simulink model "aurora1_adcs_1axis"  (R2026a)
settings: Solver=VariableStepAuto  StopTime=20.0
settings Model: Creator=chancellordelk  LastModifiedBy=chancellordelk

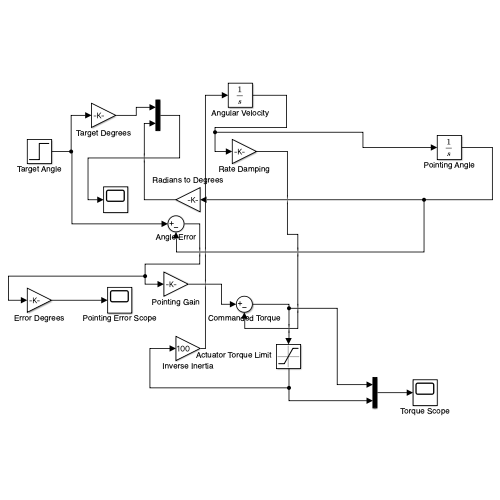
[thumbnail: Simulink's stored preview of the top-level diagram]
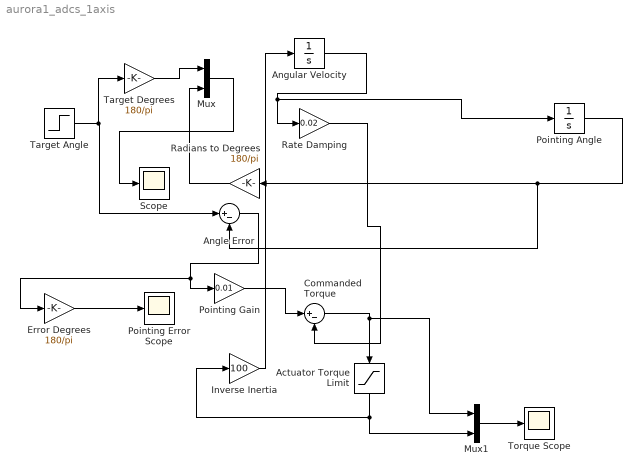
== system aurora1_adcs_1axis ==
  Actuator Torque Limit : Saturate  UpperLimit=0.0002  LowerLimit=-0.0002
  Angle Error : Sum  Inputs=|+-
  Angular Velocity : Integrator
  Commanded Torque : Sum  Inputs=|+-
  Error Degrees : Gain  Gain=180/pi
  Inverse Inertia : Gain  Gain=100
  Mux : Mux  Inputs=2
  Mux1 : Mux  Inputs=2
  Pointing Angle : Integrator
  Pointing Error Scope : Scope
      settings: ActiveDisplayYMinimum=-1.2499999999999998  ActiveDisplayYMaximum=11.25  DataLoggingVariableName=ScopeData2
  Pointing Gain : Gain  Gain=0.01
  Radians to Degrees : Gain  Gain=180/pi
  Rate Damping : Gain  Gain=0.02
  Scope : Scope
      settings: ActiveDisplayYMinimum=-1.2499999999999998  ActiveDisplayYMaximum=11.25
  Target Angle : Step  FinalValue=10*pi/180  SampleTime=0
  Target Degrees : Gain  Gain=180/pi
  Torque Scope : Scope
      settings: ActiveDisplayYMinimum=-0.00042774631399174906  ActiveDisplayYMaximum=0.0019867820926594494
  wires:
  Rate Damping/1 -> Commanded Torque/2
  Inverse Inertia/1 -> Angular Velocity/1
  Pointing Angle/1 -> Angle Error/2, Radians to Degrees/1
  Target Angle/1 -> Target Degrees/1, Angle Error/1
  Angle Error/1 -> Error Degrees/1, Pointing Gain/1
  Pointing Gain/1 -> Commanded Torque/1
  Commanded Torque/1 -> Mux1/1, Actuator Torque Limit/1
  Angular Velocity/1 -> Pointing Angle/1, Rate Damping/1
  Target Degrees/1 -> Mux/1
  Radians to Degrees/1 -> Mux/2
  Mux/1 -> Scope/1
  Actuator Torque Limit/1 -> Mux1/2, Inverse Inertia/1
  Mux1/1 -> Torque Scope/1
  Error Degrees/1 -> Pointing Error Scope/1
